simulink model "sm_car"  (R2025a)
settings: Solver=ode23t  StartTime=0.0  StopTime=400  MaxStep=0.4  RelTol=1e-3  AbsTol=1e-3  EnableMultiTasking=on
PreLoadFcn:
  | % Due to usability issue in Repeating Sequence block
  | warning('off','Simulink:Masking:Invalid');
  | 
  | % Eliminate unnecessary warnings in inactive variants
  | % Warnings generated only if you click through inactive variant
  | warning('off','MATLAB:nonExistentField');
  | warning('off','Simulink:Parameters:BlkParamUndefined');
PostLoadFcn:
  | set_param([bdroot '/Vehicle'],'popup_trailer','Off')
  | warning('off','sm:sli:setup:compile:LocalSolverNotSupported')
  | %sm_car_config_maneuver(bdroot,'WOT Braking');
  | sm_car_config_vehicle(bdroot,'false');
  | sm_car_config_logging(bdroot);
InitFcn:
  | sm_car_config_camera;
  | Vehicle = sm_car_vehcfg_checkConfig(Vehicle);
  | sm_car_check_tire_model(bdroot);
StartFcn:
  | tic;
StopFcn:
  | Elapsed_Sim_Time = toc;
  | % disp(['Elapsed Sim Time = ' num2str(Elapsed_Sim_Time)]);
undefined symbols (not defined in the file): Axle1D, AxleIn, Camera, Control, Driver, Free, Init, Maneuver, Pedal, RaceFix, RaceSpin, Scene, ShaftL1, ShaftL2, ShaftR1, ShaftR2, Soft, Stiff, Visual, X, xy_data_car_side, Y, Z
libraries: sm_lib x1546, nesl_utility x528, fl_lib x480, SimscapeFluids_lib x61, sdl_lib x49, simulink x29, ee_lib x7, simulink_extras x6, Linkage_Systems x4, Tire_1x2x x4, AntiRollBar_Systems x2, Linkage_Decoupled x2
(part 23 of 79)

== system sm_car/Vehicle/Vehicle/Chassis/Damper/Decoupled/Damper A1 Heave/Variable Endstop NL ==
  note: Sensing
  Ctrl : Inport
  Bumpstop : sdl_lib/Couplings & Drives/Springs & Dampers/Nonlinear Translational Spring  parameterization=sdl.enum.polynomialTLU.tlu  symmetry=sdl.enum.symmetry.twoSided  coefficient_vector=[100, 0, 10, 0, 1] N/m  tension_coefficient_vector=[100, 0, 10, 0, 1] N/m  compression_coefficient_vector=[1000, -10, 100, 0, 0] N/m  deformation_vector=xEndstop m  force_vector=fEndstop N  interp_method=simscape.enum.interpolation.linear  extrap_method=simscape.enum.extrapolation.linear  x_specify=on  x_priority=None  x=0 m  x_nominal_specify=off  x_nominal_value=1  x_nominal_unit=m
      settings: InternalSimscapePortConfiguration="{\"Bottom\":[],\"Left\":[{\"id\":\"R\",\"label\":\"R\",\"type\":\"foundation.mechanical.translational.translational\"}],\"Right\":[{\"id\":\"C\",\"label\":\"C\",\"type\":\"foundation.mechanical.translational.translational\"}],\"Top\":[]}"
  Damper : sdl_lib/Couplings & Drives/Springs & Dampers/Variable Translational Damper  Bmin=0 N*s/m
      settings: InternalSimscapePortConfiguration="{\"Bottom\":[],\"Left\":[{\"id\":\"B\",\"label\":\"B\",\"type\":\"input\"},{\"id\":\"R\",\"label\":\"R\",\"type\":\"foundation.mechanical.translational.translational\"}],\"Right\":[{\"id\":\"C\",\"label\":\"C\",\"type\":\"foundation.mechanical.translational.translational\"}],\"Top\":[]}"
  Force Bumpstop : fl_lib/Mechanical/Mechanical Sensors/Ideal Force Sensor
  Force Damper : fl_lib/Mechanical/Mechanical Sensors/Ideal Force Sensor
  Motion Damper : fl_lib/Mechanical/Mechanical Sensors/Ideal Translational Motion Sensor  reference=foundation.enum.MeasurementReference.difference  acceleration_port=false  velocity_port=true  position_port=true  offset=dam_x0 m
  PS-Simulink Converter : nesl_utility/PS-Simulink Converter  PhysicalDomain=network_engine_domain  SubClassName=ps_output  LeftPortType=input  RightPortType=output  PseudoPeriodic=off  Frequencies=[]  VectorFormat=1-D array  Unit=N  AffineConversion=off
  PS-Simulink Converter1 : nesl_utility/PS-Simulink Converter  PhysicalDomain=network_engine_domain  SubClassName=ps_output  LeftPortType=input  RightPortType=output  PseudoPeriodic=off  Frequencies=[]  VectorFormat=1-D array  Unit=N  AffineConversion=off
  PS-Simulink Converter2 : nesl_utility/PS-Simulink Converter  PhysicalDomain=network_engine_domain  SubClassName=ps_output  LeftPortType=input  RightPortType=output  PseudoPeriodic=off  Frequencies=[]  VectorFormat=1-D array  Unit=m/s  AffineConversion=off
  PS-Simulink Converter3 : nesl_utility/PS-Simulink Converter  PhysicalDomain=network_engine_domain  SubClassName=ps_output  LeftPortType=input  RightPortType=output  PseudoPeriodic=off  Frequencies=[]  VectorFormat=1-D array  Unit=m  AffineConversion=off
  Simulink-PS Converter : nesl_utility/Simulink-PS Converter  PhysicalDomain=network_engine_domain  SubClassName=ps_input  LeftPortType=input  RightPortType=output  PseudoPeriodic=off  Frequencies=[]  NoiseDistribution=none  NoiseParameters=[]  Unit=N*s/m  AffineConversion=off  FilteringAndDerivatives=provide  SimscapeFilterOrder=1  InputFilterTimeConstant=0.001  UdotUserProvided=0
  R : PMIOPort  Side=Left
  C : PMIOPort  Port=2  Side=Right
  Out Bus Element : Outport  VectorParamsAs1DForOutWhenUnconnected=off  PortName=meas  Element=FDamper
  Out Bus Element1 : Outport  VectorParamsAs1DForOutWhenUnconnected=off  PortName=meas  Element=FBumpstop
  Out Bus Element2 : Outport  VectorParamsAs1DForOutWhenUnconnected=off  PortName=meas  Element=xDamper
  Out Bus Element3 : Outport  VectorParamsAs1DForOutWhenUnconnected=off  PortName=meas  Element=vDamper
  wires:
  PS-Simulink Converter1/1 -> Out Bus Element1/1
  PS-Simulink Converter3/1 -> Out Bus Element2/1
  PS-Simulink Converter2/1 -> Out Bus Element3/1
  PS-Simulink Converter/1 -> Out Bus Element/1
  Ctrl/1 -> Simulink-PS Converter/1
  connections:
  Simulink-PS Converter/RConn1 -- Damper/LConn1
  R/RConn1 -- Motion Damper/LConn1 -- Bumpstop/LConn1 -- Damper/LConn2
  Force Damper/RConn1 -- Damper/RConn1
  Bumpstop/RConn1 -- Force Bumpstop/RConn1
  PS-Simulink Converter/LConn1 -- Force Damper/RConn2
  PS-Simulink Converter3/LConn1 -- Motion Damper/RConn3
  PS-Simulink Converter1/LConn1 -- Force Bumpstop/RConn2
  PS-Simulink Converter2/LConn1 -- Motion Damper/RConn2
  Force Damper/LConn1 -- C/RConn1 -- Force Bumpstop/LConn1 -- Motion Damper/RConn1

== system sm_car/Vehicle/Vehicle/Chassis/Damper/Decoupled/Damper A1 Roll/Force Endstop NL ==
  note: Sensing
  Ctrl : Inport
  Bumpstop : sdl_lib/Couplings & Drives/Springs & Dampers/Nonlinear Translational Spring  parameterization=sdl.enum.polynomialTLU.tlu  symmetry=sdl.enum.symmetry.twoSided  coefficient_vector=[100, 0, 10, 0, 1] N/m  tension_coefficient_vector=[100, 0, 10, 0, 1] N/m  compression_coefficient_vector=[1000, -10, 100, 0, 0] N/m  deformation_vector=xEndstop m  force_vector=fEndstop N  interp_method=simscape.enum.interpolation.linear  extrap_method=simscape.enum.extrapolation.linear  x_specify=on  x_priority=None  x=0 m  x_nominal_specify=off  x_nominal_value=1  x_nominal_unit=m
      settings: InternalSimscapePortConfiguration="{\"Bottom\":[],\"Left\":[{\"id\":\"R\",\"label\":\"R\",\"type\":\"foundation.mechanical.translational.translational\"}],\"Right\":[{\"id\":\"C\",\"label\":\"C\",\"type\":\"foundation.mechanical.translational.translational\"}],\"Top\":[]}"
  Force Source : fl_lib/Mechanical/Mechanical Sources/Ideal Force Source
  Force Bumpstop : fl_lib/Mechanical/Mechanical Sensors/Ideal Force Sensor
  Force Damper : fl_lib/Mechanical/Mechanical Sensors/Ideal Force Sensor
  Motion Damper : fl_lib/Mechanical/Mechanical Sensors/Ideal Translational Motion Sensor  reference=foundation.enum.MeasurementReference.difference  acceleration_port=false  velocity_port=true  position_port=true  offset=dam_x0 m
  PS-Simulink Converter : nesl_utility/PS-Simulink Converter  PhysicalDomain=network_engine_domain  SubClassName=ps_output  LeftPortType=input  RightPortType=output  PseudoPeriodic=off  Frequencies=[]  VectorFormat=1-D array  Unit=N  AffineConversion=off
  PS-Simulink Converter1 : nesl_utility/PS-Simulink Converter  PhysicalDomain=network_engine_domain  SubClassName=ps_output  LeftPortType=input  RightPortType=output  PseudoPeriodic=off  Frequencies=[]  VectorFormat=1-D array  Unit=N  AffineConversion=off
  PS-Simulink Converter2 : nesl_utility/PS-Simulink Converter  PhysicalDomain=network_engine_domain  SubClassName=ps_output  LeftPortType=input  RightPortType=output  PseudoPeriodic=off  Frequencies=[]  VectorFormat=1-D array  Unit=m/s  AffineConversion=off
  PS-Simulink Converter3 : nesl_utility/PS-Simulink Converter  PhysicalDomain=network_engine_domain  SubClassName=ps_output  LeftPortType=input  RightPortType=output  PseudoPeriodic=off  Frequencies=[]  VectorFormat=1-D array  Unit=m  AffineConversion=off
  Simulink-PS Converter : nesl_utility/Simulink-PS Converter  PhysicalDomain=network_engine_domain  SubClassName=ps_input  LeftPortType=input  RightPortType=output  PseudoPeriodic=off  Frequencies=[]  NoiseDistribution=none  NoiseParameters=[]  Unit=N  AffineConversion=off  FilteringAndDerivatives=filter  SimscapeFilterOrder=1  InputFilterTimeConstant=0.01  UdotUserProvided=0
  R : PMIOPort  Side=Left
  C : PMIOPort  Port=2  Side=Right
  Out Bus Element : Outport  VectorParamsAs1DForOutWhenUnconnected=off  PortName=meas  Element=FDamper
  Out Bus Element1 : Outport  VectorParamsAs1DForOutWhenUnconnected=off  PortName=meas  Element=FBumpstop
  Out Bus Element2 : Outport  VectorParamsAs1DForOutWhenUnconnected=off  PortName=meas  Element=xDamper
  Out Bus Element3 : Outport  VectorParamsAs1DForOutWhenUnconnected=off  PortName=meas  Element=vDamper
  wires:
  PS-Simulink Converter1/1 -> Out Bus Element1/1
  PS-Simulink Converter3/1 -> Out Bus Element2/1
  PS-Simulink Converter2/1 -> Out Bus Element3/1
  PS-Simulink Converter/1 -> Out Bus Element/1
  Ctrl/1 -> Simulink-PS Converter/1
  connections:
  Simulink-PS Converter/RConn1 -- Force Source/RConn1
  Force Source/RConn2 -- Bumpstop/LConn1 -- R/RConn1 -- Motion Damper/LConn1
  Force Source/LConn1 -- Force Damper/RConn1
  Bumpstop/RConn1 -- Force Bumpstop/RConn1
  PS-Simulink Converter/LConn1 -- Force Damper/RConn2
  PS-Simulink Converter3/LConn1 -- Motion Damper/RConn3
  PS-Simulink Converter1/LConn1 -- Force Bumpstop/RConn2
  PS-Simulink Converter2/LConn1 -- Motion Damper/RConn2
  Force Damper/LConn1 -- C/RConn1 -- Force Bumpstop/LConn1 -- Motion Damper/RConn1

== system sm_car/Vehicle/Vehicle/Chassis/Damper/Decoupled/Damper A1 Roll/Linear ==
  note: Sensing
  Ctrl : Inport
  Bumpstop : fl_lib/Mechanical/Translational Elements/Translational Hard Stop  upper_bnd=bs_lim_upper m  lower_bnd=bs_lim_lower m  model=1  stiff_up=bs_k_upper N/m  stiff_low=bs_k_lower N/m  D_up=bs_b_upper N/(m/s)  D_low=bs_b_lower N/(m/s)  transition=bs_region m  coeff_rest=0.7  v_tol=0.001 m/s  f_tol=0.001 N  v_specify=off  v_priority=None  v=0 m/s  v_nominal_specify=off  v_nominal_value=1  v_nominal_unit=m/s  f_specify=off  f_priority=None  f=0 N  f_nominal_specify=off  f_nominal_value=1  f_nominal_unit=N  x_specify=off  x_priority=High  x=0 m  x_nominal_specify=off  x_nominal_value=1  x_nominal_unit=m  M_specify=off  M_priority=None  M=0
  Damper : fl_lib/Mechanical/Translational Elements/Translational Damper  D=dam_b N/(m/s)  v_specify=off  v_priority=None  v=0 m/s  v_nominal_specify=off  v_nominal_value=1  v_nominal_unit=m/s  f_specify=off  f_priority=None  f=0 N  f_nominal_specify=off  f_nominal_value=1  f_nominal_unit=N
  Force Bumpstop : fl_lib/Mechanical/Mechanical Sensors/Ideal Force Sensor
  Force Damper : fl_lib/Mechanical/Mechanical Sensors/Ideal Force Sensor
  Motion Damper : fl_lib/Mechanical/Mechanical Sensors/Ideal Translational Motion Sensor  reference=foundation.enum.MeasurementReference.difference  acceleration_port=false  velocity_port=true  position_port=true  offset=dam_x0 m
  PS-Simulink Converter : nesl_utility/PS-Simulink Converter  PhysicalDomain=network_engine_domain  SubClassName=ps_output  LeftPortType=input  RightPortType=output  PseudoPeriodic=off  Frequencies=[]  VectorFormat=1-D array  Unit=N  AffineConversion=off
  PS-Simulink Converter1 : nesl_utility/PS-Simulink Converter  PhysicalDomain=network_engine_domain  SubClassName=ps_output  LeftPortType=input  RightPortType=output  PseudoPeriodic=off  Frequencies=[]  VectorFormat=1-D array  Unit=N  AffineConversion=off
  PS-Simulink Converter2 : nesl_utility/PS-Simulink Converter  PhysicalDomain=network_engine_domain  SubClassName=ps_output  LeftPortType=input  RightPortType=output  PseudoPeriodic=off  Frequencies=[]  VectorFormat=1-D array  Unit=m/s  AffineConversion=off
  PS-Simulink Converter3 : nesl_utility/PS-Simulink Converter  PhysicalDomain=network_engine_domain  SubClassName=ps_output  LeftPortType=input  RightPortType=output  PseudoPeriodic=off  Frequencies=[]  VectorFormat=1-D array  Unit=m  AffineConversion=off
  Terminator : Terminator
  R : PMIOPort  Side=Left
  C : PMIOPort  Port=2  Side=Right
  Out Bus Element : Outport  VectorParamsAs1DForOutWhenUnconnected=off  PortName=meas  Element=FDamper
  Out Bus Element1 : Outport  VectorParamsAs1DForOutWhenUnconnected=off  PortName=meas  Element=FBumpstop
  Out Bus Element2 : Outport  VectorParamsAs1DForOutWhenUnconnected=off  PortName=meas  Element=xDamper
  Out Bus Element3 : Outport  VectorParamsAs1DForOutWhenUnconnected=off  PortName=meas  Element=vDamper
  wires:
  PS-Simulink Converter1/1 -> Out Bus Element1/1
  PS-Simulink Converter3/1 -> Out Bus Element2/1
  PS-Simulink Converter2/1 -> Out Bus Element3/1
  PS-Simulink Converter/1 -> Out Bus Element/1
  Ctrl/1 -> Terminator/1
  connections:
  R/RConn1 -- Motion Damper/LConn1 -- Bumpstop/LConn1 -- Damper/LConn1
  Force Damper/RConn1 -- Damper/RConn1
  Force Bumpstop/RConn1 -- Bumpstop/RConn1
  PS-Simulink Converter/LConn1 -- Force Damper/RConn2
  PS-Simulink Converter3/LConn1 -- Motion Damper/RConn3
  PS-Simulink Converter1/LConn1 -- Force Bumpstop/RConn2
  PS-Simulink Converter2/LConn1 -- Motion Damper/RConn2
  Force Damper/LConn1 -- C/RConn1 -- Force Bumpstop/LConn1 -- Motion Damper/RConn1

== system sm_car/Vehicle/Vehicle/Chassis/Damper/Decoupled/Damper A1 Roll/None ==
  note: Sensor inserted simply to ensure
      | all blocks are connected to a network
  Ctrl : Inport
  Constant{1..4} (4 alike) : Constant  Value=0
  Ideal Translational Motion Sensor : fl_lib/Mechanical/Mechanical Sensors/Ideal Translational Motion Sensor  reference=foundation.enum.MeasurementReference.difference  acceleration_port=false  velocity_port=true  position_port=true  offset=0 m
  PS-Simulink Converter2 : nesl_utility/PS-Simulink Converter  PhysicalDomain=network_engine_domain  SubClassName=ps_output  LeftPortType=input  RightPortType=output  PseudoPeriodic=off  Frequencies=[]  VectorFormat=1-D array  Unit=1  AffineConversion=off
  PS-Simulink Converter3 : nesl_utility/PS-Simulink Converter  PhysicalDomain=network_engine_domain  SubClassName=ps_output  LeftPortType=input  RightPortType=output  PseudoPeriodic=off  Frequencies=[]  VectorFormat=1-D array  Unit=1  AffineConversion=off
  Terminator : Terminator
  Terminator1 : Terminator
  Terminator2 : Terminator
  R : PMIOPort  Side=Left
  C : PMIOPort  Port=2  Side=Right
  Out Bus Element : Outport  VectorParamsAs1DForOutWhenUnconnected=off  PortName=meas  Element=FDamper
  Out Bus Element1 : Outport  VectorParamsAs1DForOutWhenUnconnected=off  PortName=meas  Element=FBumpstop
  Out Bus Element2 : Outport  VectorParamsAs1DForOutWhenUnconnected=off  PortName=meas  Element=xDamper
  Out Bus Element3 : Outport  VectorParamsAs1DForOutWhenUnconnected=off  PortName=meas  Element=vDamper
  wires:
  PS-Simulink Converter2/1 -> Terminator1/1
  PS-Simulink Converter3/1 -> Terminator2/1
  Constant2/1 -> Out Bus Element1/1
  Constant4/1 -> Out Bus Element2/1
  Constant3/1 -> Out Bus Element3/1
  Constant1/1 -> Out Bus Element/1
  Ctrl/1 -> Terminator/1
  connections:
  C/RConn1 -- Ideal Translational Motion Sensor/RConn1
  R/RConn1 -- Ideal Translational Motion Sensor/LConn1
  PS-Simulink Converter3/LConn1 -- Ideal Translational Motion Sensor/RConn3
  Ideal Translational Motion Sensor/RConn2 -- PS-Simulink Converter2/LConn1

== system sm_car/Vehicle/Vehicle/Chassis/Damper/Decoupled/Damper A1 Roll/Nonlinear ==
  note: Sensing
  Ctrl : Inport
  Bumpstop : fl_lib/Mechanical/Translational Elements/Translational Hard Stop  upper_bnd=bs_lim_upper m  lower_bnd=bs_lim_lower m  model=1  stiff_up=bs_k_upper N/m  stiff_low=bs_k_lower N/m  D_up=bs_b_upper N/(m/s)  D_low=bs_b_lower N/(m/s)  transition=bs_region m  coeff_rest=0.7  v_tol=0.001 m/s  f_tol=0.001 N  v_specify=off  v_priority=None  v=0 m/s  v_nominal_specify=off  v_nominal_value=1  v_nominal_unit=m/s  f_specify=off  f_priority=None  f=0 N  f_nominal_specify=off  f_nominal_value=1  f_nominal_unit=N  x_specify=off  x_priority=High  x=0 m  x_nominal_specify=off  x_nominal_value=1  x_nominal_unit=m  M_specify=off  M_priority=None  M=0
  Damper : sdl_lib/Couplings & Drives/Springs & Dampers/Nonlinear Translational Damper  parameterization=2  symmetry=1  coefficient_vector=[10, 0, 1, 0, .1] N/(m/s)  extension_coefficient_vector=[10, 0, 1, 0, .1] N/(m/s)  contraction_coefficient_vector=[100, -1, 10, 0, 0] N/(m/s)  velocity_vector=velocity_vector m/s  force_vector=force_vector N  interp_method=simscape.enum.interpolation.linear  extrap_method=simscape.enum.extrapolation.linear
      settings: InternalSimscapePortConfiguration="{\"Bottom\":[],\"Left\":[{\"id\":\"R\",\"label\":\"R\",\"type\":\"foundation.mechanical.translational.translational\"}],\"Right\":[{\"id\":\"C\",\"label\":\"C\",\"type\":\"foundation.mechanical.translational.translational\"}],\"Top\":[]}"
  Force Bumpstop : fl_lib/Mechanical/Mechanical Sensors/Ideal Force Sensor
  Force Damper : fl_lib/Mechanical/Mechanical Sensors/Ideal Force Sensor
  Motion Damper : fl_lib/Mechanical/Mechanical Sensors/Ideal Translational Motion Sensor  reference=foundation.enum.MeasurementReference.difference  acceleration_port=false  velocity_port=true  position_port=true  offset=dam_x0 m
  PS-Simulink Converter : nesl_utility/PS-Simulink Converter  PhysicalDomain=network_engine_domain  SubClassName=ps_output  LeftPortType=input  RightPortType=output  PseudoPeriodic=off  Frequencies=[]  VectorFormat=1-D array  Unit=N  AffineConversion=off
  PS-Simulink Converter1 : nesl_utility/PS-Simulink Converter  PhysicalDomain=network_engine_domain  SubClassName=ps_output  LeftPortType=input  RightPortType=output  PseudoPeriodic=off  Frequencies=[]  VectorFormat=1-D array  Unit=N  AffineConversion=off
  PS-Simulink Converter2 : nesl_utility/PS-Simulink Converter  PhysicalDomain=network_engine_domain  SubClassName=ps_output  LeftPortType=input  RightPortType=output  PseudoPeriodic=off  Frequencies=[]  VectorFormat=1-D array  Unit=m/s  AffineConversion=off
  PS-Simulink Converter3 : nesl_utility/PS-Simulink Converter  PhysicalDomain=network_engine_domain  SubClassName=ps_output  LeftPortType=input  RightPortType=output  PseudoPeriodic=off  Frequencies=[]  VectorFormat=1-D array  Unit=m  AffineConversion=off
  Terminator : Terminator
  R : PMIOPort  Side=Left
  C : PMIOPort  Port=2  Side=Right
  Out Bus Element : Outport  VectorParamsAs1DForOutWhenUnconnected=off  PortName=meas  Element=FDamper
  Out Bus Element1 : Outport  VectorParamsAs1DForOutWhenUnconnected=off  PortName=meas  Element=FBumpstop
  Out Bus Element2 : Outport  VectorParamsAs1DForOutWhenUnconnected=off  PortName=meas  Element=xDamper
  Out Bus Element3 : Outport  VectorParamsAs1DForOutWhenUnconnected=off  PortName=meas  Element=vDamper
  wires:
  Ctrl/1 -> Terminator/1
  PS-Simulink Converter/1 -> Out Bus Element/1
  PS-Simulink Converter2/1 -> Out Bus Element3/1
  PS-Simulink Converter3/1 -> Out Bus Element2/1
  PS-Simulink Converter1/1 -> Out Bus Element1/1
  connections:
  Motion Damper/RConn1 -- Force Bumpstop/LConn1 -- C/RConn1 -- Force Damper/LConn1
  PS-Simulink Converter2/LConn1 -- Motion Damper/RConn2
  PS-Simulink Converter1/LConn1 -- Force Bumpstop/RConn2
  PS-Simulink Converter3/LConn1 -- Motion Damper/RConn3
  PS-Simulink Converter/LConn1 -- Force Damper/RConn2
  Force Bumpstop/RConn1 -- Bumpstop/RConn1
  Damper/RConn1 -- Force Damper/RConn1
  Bumpstop/LConn1 -- Motion Damper/LConn1 -- R/RConn1 -- Damper/LConn1

== system sm_car/Vehicle/Vehicle/Chassis/Damper/Decoupled/Damper A1 Roll/Nonlinear Endstop NL ==
  note: Sensing
  Ctrl : Inport
  Bumpstop : sdl_lib/Couplings & Drives/Springs & Dampers/Nonlinear Translational Spring  parameterization=sdl.enum.polynomialTLU.tlu  symmetry=sdl.enum.symmetry.twoSided  coefficient_vector=[100, 0, 10, 0, 1] N/m  tension_coefficient_vector=[100, 0, 10, 0, 1] N/m  compression_coefficient_vector=[1000, -10, 100, 0, 0] N/m  deformation_vector=xEndstop m  force_vector=fEndstop N  interp_method=simscape.enum.interpolation.linear  extrap_method=simscape.enum.extrapolation.linear  x_specify=on  x_priority=None  x=0 m  x_nominal_specify=off  x_nominal_value=1  x_nominal_unit=m
      settings: InternalSimscapePortConfiguration="{\"Bottom\":[],\"Left\":[{\"id\":\"R\",\"label\":\"R\",\"type\":\"foundation.mechanical.translational.translational\"}],\"Right\":[{\"id\":\"C\",\"label\":\"C\",\"type\":\"foundation.mechanical.translational.translational\"}],\"Top\":[]}"
  Damper : sdl_lib/Couplings & Drives/Springs & Dampers/Nonlinear Translational Damper  parameterization=2  symmetry=1  coefficient_vector=[10, 0, 1, 0, .1] N/(m/s)  extension_coefficient_vector=[10, 0, 1, 0, .1] N/(m/s)  contraction_coefficient_vector=[100, -1, 10, 0, 0] N/(m/s)  velocity_vector=velocity_vector m/s  force_vector=force_vector N  interp_method=simscape.enum.interpolation.linear  extrap_method=simscape.enum.extrapolation.linear
      settings: InternalSimscapePortConfiguration="{\"Bottom\":[],\"Left\":[{\"id\":\"R\",\"label\":\"R\",\"type\":\"foundation.mechanical.translational.translational\"}],\"Right\":[{\"id\":\"C\",\"label\":\"C\",\"type\":\"foundation.mechanical.translational.translational\"}],\"Top\":[]}"
  Force Bumpstop : fl_lib/Mechanical/Mechanical Sensors/Ideal Force Sensor
  Force Damper : fl_lib/Mechanical/Mechanical Sensors/Ideal Force Sensor
  Motion Damper : fl_lib/Mechanical/Mechanical Sensors/Ideal Translational Motion Sensor  reference=foundation.enum.MeasurementReference.difference  acceleration_port=false  velocity_port=true  position_port=true  offset=dam_x0 m
  PS-Simulink Converter : nesl_utility/PS-Simulink Converter  PhysicalDomain=network_engine_domain  SubClassName=ps_output  LeftPortType=input  RightPortType=output  PseudoPeriodic=off  Frequencies=[]  VectorFormat=1-D array  Unit=N  AffineConversion=off
  PS-Simulink Converter1 : nesl_utility/PS-Simulink Converter  PhysicalDomain=network_engine_domain  SubClassName=ps_output  LeftPortType=input  RightPortType=output  PseudoPeriodic=off  Frequencies=[]  VectorFormat=1-D array  Unit=N  AffineConversion=off
  PS-Simulink Converter2 : nesl_utility/PS-Simulink Converter  PhysicalDomain=network_engine_domain  SubClassName=ps_output  LeftPortType=input  RightPortType=output  PseudoPeriodic=off  Frequencies=[]  VectorFormat=1-D array  Unit=m/s  AffineConversion=off
  PS-Simulink Converter3 : nesl_utility/PS-Simulink Converter  PhysicalDomain=network_engine_domain  SubClassName=ps_output  LeftPortType=input  RightPortType=output  PseudoPeriodic=off  Frequencies=[]  VectorFormat=1-D array  Unit=m  AffineConversion=off
  Terminator : Terminator
  R : PMIOPort  Side=Left
  C : PMIOPort  Port=2  Side=Right
  Out Bus Element : Outport  VectorParamsAs1DForOutWhenUnconnected=off  PortName=meas  Element=FDamper
  Out Bus Element1 : Outport  VectorParamsAs1DForOutWhenUnconnected=off  PortName=meas  Element=FBumpstop
  Out Bus Element2 : Outport  VectorParamsAs1DForOutWhenUnconnected=off  PortName=meas  Element=xDamper
  Out Bus Element3 : Outport  VectorParamsAs1DForOutWhenUnconnected=off  PortName=meas  Element=vDamper
  wires:
  Ctrl/1 -> Terminator/1
  PS-Simulink Converter/1 -> Out Bus Element/1
  PS-Simulink Converter2/1 -> Out Bus Element3/1
  PS-Simulink Converter3/1 -> Out Bus Element2/1
  PS-Simulink Converter1/1 -> Out Bus Element1/1
  connections:
  Motion Damper/RConn1 -- Force Bumpstop/LConn1 -- C/RConn1 -- Force Damper/LConn1
  PS-Simulink Converter2/LConn1 -- Motion Damper/RConn2
  PS-Simulink Converter1/LConn1 -- Force Bumpstop/RConn2
  PS-Simulink Converter3/LConn1 -- Motion Damper/RConn3
  PS-Simulink Converter/LConn1 -- Force Damper/RConn2
  Force Bumpstop/RConn1 -- Bumpstop/RConn1
  Damper/RConn1 -- Force Damper/RConn1
  Motion Damper/LConn1 -- R/RConn1 -- Bumpstop/LConn1 -- Damper/LConn1

== system sm_car/Vehicle/Vehicle/Chassis/Damper/Decoupled/Damper A1 Roll/Variable ==
  note: Sensing
  Ctrl : Inport
  Bumpstop : fl_lib/Mechanical/Translational Elements/Translational Hard Stop  upper_bnd=bs_lim_upper m  lower_bnd=bs_lim_lower m  model=1  stiff_up=bs_k_upper N/m  stiff_low=bs_k_lower N/m  D_up=bs_b_upper N/(m/s)  D_low=bs_b_lower N/(m/s)  transition=bs_region m  coeff_rest=0.7  v_tol=0.001 m/s  f_tol=0.001 N  v_specify=off  v_priority=None  v=0 m/s  v_nominal_specify=off  v_nominal_value=1  v_nominal_unit=m/s  f_specify=off  f_priority=None  f=0 N  f_nominal_specify=off  f_nominal_value=1  f_nominal_unit=N  x_specify=off  x_priority=High  x=0 m  x_nominal_specify=off  x_nominal_value=1  x_nominal_unit=m  M_specify=off  M_priority=None  M=0
  Damper : sdl_lib/Couplings & Drives/Springs & Dampers/Variable Translational Damper  Bmin=0 N*s/m
      settings: InternalSimscapePortConfiguration="{\"Bottom\":[],\"Left\":[{\"id\":\"B\",\"label\":\"B\",\"type\":\"input\"},{\"id\":\"R\",\"label\":\"R\",\"type\":\"foundation.mechanical.translational.translational\"}],\"Right\":[{\"id\":\"C\",\"label\":\"C\",\"type\":\"foundation.mechanical.translational.translational\"}],\"Top\":[]}"
  Force Bumpstop : fl_lib/Mechanical/Mechanical Sensors/Ideal Force Sensor
  Force Damper : fl_lib/Mechanical/Mechanical Sensors/Ideal Force Sensor
  Motion Damper : fl_lib/Mechanical/Mechanical Sensors/Ideal Translational Motion Sensor  reference=foundation.enum.MeasurementReference.difference  acceleration_port=false  velocity_port=true  position_port=true  offset=dam_x0 m
  PS-Simulink Converter : nesl_utility/PS-Simulink Converter  PhysicalDomain=network_engine_domain  SubClassName=ps_output  LeftPortType=input  RightPortType=output  PseudoPeriodic=off  Frequencies=[]  VectorFormat=1-D array  Unit=N  AffineConversion=off
  PS-Simulink Converter1 : nesl_utility/PS-Simulink Converter  PhysicalDomain=network_engine_domain  SubClassName=ps_output  LeftPortType=input  RightPortType=output  PseudoPeriodic=off  Frequencies=[]  VectorFormat=1-D array  Unit=N  AffineConversion=off
  PS-Simulink Converter2 : nesl_utility/PS-Simulink Converter  PhysicalDomain=network_engine_domain  SubClassName=ps_output  LeftPortType=input  RightPortType=output  PseudoPeriodic=off  Frequencies=[]  VectorFormat=1-D array  Unit=m/s  AffineConversion=off
  PS-Simulink Converter3 : nesl_utility/PS-Simulink Converter  PhysicalDomain=network_engine_domain  SubClassName=ps_output  LeftPortType=input  RightPortType=output  PseudoPeriodic=off  Frequencies=[]  VectorFormat=1-D array  Unit=m  AffineConversion=off
  Simulink-PS Converter : nesl_utility/Simulink-PS Converter  PhysicalDomain=network_engine_domain  SubClassName=ps_input  LeftPortType=input  RightPortType=output  PseudoPeriodic=off  Frequencies=[]  NoiseDistribution=none  NoiseParameters=[]  Unit=N*s/m  AffineConversion=off  FilteringAndDerivatives=provide  SimscapeFilterOrder=1  InputFilterTimeConstant=0.001  UdotUserProvided=0
  R : PMIOPort  Side=Left
  C : PMIOPort  Port=2  Side=Right
  Out Bus Element : Outport  VectorParamsAs1DForOutWhenUnconnected=off  PortName=meas  Element=FDamper
  Out Bus Element1 : Outport  VectorParamsAs1DForOutWhenUnconnected=off  PortName=meas  Element=FBumpstop
  Out Bus Element2 : Outport  VectorParamsAs1DForOutWhenUnconnected=off  PortName=meas  Element=xDamper
  Out Bus Element3 : Outport  VectorParamsAs1DForOutWhenUnconnected=off  PortName=meas  Element=vDamper
  wires:
  PS-Simulink Converter1/1 -> Out Bus Element1/1
  PS-Simulink Converter3/1 -> Out Bus Element2/1
  PS-Simulink Converter2/1 -> Out Bus Element3/1
  PS-Simulink Converter/1 -> Out Bus Element/1
  Ctrl/1 -> Simulink-PS Converter/1
  connections:
  Simulink-PS Converter/RConn1 -- Damper/LConn1
  R/RConn1 -- Motion Damper/LConn1 -- Damper/LConn2 -- Bumpstop/LConn1
  Force Damper/RConn1 -- Damper/RConn1
  Force Bumpstop/RConn1 -- Bumpstop/RConn1
  PS-Simulink Converter/LConn1 -- Force Damper/RConn2
  PS-Simulink Converter3/LConn1 -- Motion Damper/RConn3
  PS-Simulink Converter1/LConn1 -- Force Bumpstop/RConn2
  PS-Simulink Converter2/LConn1 -- Motion Damper/RConn2
  Force Damper/LConn1 -- C/RConn1 -- Force Bumpstop/LConn1 -- Motion Damper/RConn1

== system sm_car/Vehicle/Vehicle/Chassis/Damper/Decoupled/Damper A1 Roll/Variable Endstop NL ==
  note: Sensing
  Ctrl : Inport
  Bumpstop : sdl_lib/Couplings & Drives/Springs & Dampers/Nonlinear Translational Spring  parameterization=sdl.enum.polynomialTLU.tlu  symmetry=sdl.enum.symmetry.twoSided  coefficient_vector=[100, 0, 10, 0, 1] N/m  tension_coefficient_vector=[100, 0, 10, 0, 1] N/m  compression_coefficient_vector=[1000, -10, 100, 0, 0] N/m  deformation_vector=xEndstop m  force_vector=fEndstop N  interp_method=simscape.enum.interpolation.linear  extrap_method=simscape.enum.extrapolation.linear  x_specify=on  x_priority=None  x=0 m  x_nominal_specify=off  x_nominal_value=1  x_nominal_unit=m
      settings: InternalSimscapePortConfiguration="{\"Bottom\":[],\"Left\":[{\"id\":\"R\",\"label\":\"R\",\"type\":\"foundation.mechanical.translational.translational\"}],\"Right\":[{\"id\":\"C\",\"label\":\"C\",\"type\":\"foundation.mechanical.translational.translational\"}],\"Top\":[]}"
  Damper : sdl_lib/Couplings & Drives/Springs & Dampers/Variable Translational Damper  Bmin=0 N*s/m
      settings: InternalSimscapePortConfiguration="{\"Bottom\":[],\"Left\":[{\"id\":\"B\",\"label\":\"B\",\"type\":\"input\"},{\"id\":\"R\",\"label\":\"R\",\"type\":\"foundation.mechanical.translational.translational\"}],\"Right\":[{\"id\":\"C\",\"label\":\"C\",\"type\":\"foundation.mechanical.translational.translational\"}],\"Top\":[]}"
  Force Bumpstop : fl_lib/Mechanical/Mechanical Sensors/Ideal Force Sensor
  Force Damper : fl_lib/Mechanical/Mechanical Sensors/Ideal Force Sensor
  Motion Damper : fl_lib/Mechanical/Mechanical Sensors/Ideal Translational Motion Sensor  reference=foundation.enum.MeasurementReference.difference  acceleration_port=false  velocity_port=true  position_port=true  offset=dam_x0 m
  PS-Simulink Converter : nesl_utility/PS-Simulink Converter  PhysicalDomain=network_engine_domain  SubClassName=ps_output  LeftPortType=input  RightPortType=output  PseudoPeriodic=off  Frequencies=[]  VectorFormat=1-D array  Unit=N  AffineConversion=off
  PS-Simulink Converter1 : nesl_utility/PS-Simulink Converter  PhysicalDomain=network_engine_domain  SubClassName=ps_output  LeftPortType=input  RightPortType=output  PseudoPeriodic=off  Frequencies=[]  VectorFormat=1-D array  Unit=N  AffineConversion=off
  PS-Simulink Converter2 : nesl_utility/PS-Simulink Converter  PhysicalDomain=network_engine_domain  SubClassName=ps_output  LeftPortType=input  RightPortType=output  PseudoPeriodic=off  Frequencies=[]  VectorFormat=1-D array  Unit=m/s  AffineConversion=off
  PS-Simulink Converter3 : nesl_utility/PS-Simulink Converter  PhysicalDomain=network_engine_domain  SubClassName=ps_output  LeftPortType=input  RightPortType=output  PseudoPeriodic=off  Frequencies=[]  VectorFormat=1-D array  Unit=m  AffineConversion=off
  Simulink-PS Converter : nesl_utility/Simulink-PS Converter  PhysicalDomain=network_engine_domain  SubClassName=ps_input  LeftPortType=input  RightPortType=output  PseudoPeriodic=off  Frequencies=[]  NoiseDistribution=none  NoiseParameters=[]  Unit=N*s/m  AffineConversion=off  FilteringAndDerivatives=provide  SimscapeFilterOrder=1  InputFilterTimeConstant=0.001  UdotUserProvided=0
  R : PMIOPort  Side=Left
  C : PMIOPort  Port=2  Side=Right
  Out Bus Element : Outport  VectorParamsAs1DForOutWhenUnconnected=off  PortName=meas  Element=FDamper
  Out Bus Element1 : Outport  VectorParamsAs1DForOutWhenUnconnected=off  PortName=meas  Element=FBumpstop
  Out Bus Element2 : Outport  VectorParamsAs1DForOutWhenUnconnected=off  PortName=meas  Element=xDamper
  Out Bus Element3 : Outport  VectorParamsAs1DForOutWhenUnconnected=off  PortName=meas  Element=vDamper
  wires:
  PS-Simulink Converter1/1 -> Out Bus Element1/1
  PS-Simulink Converter3/1 -> Out Bus Element2/1
  PS-Simulink Converter2/1 -> Out Bus Element3/1
  PS-Simulink Converter/1 -> Out Bus Element/1
  Ctrl/1 -> Simulink-PS Converter/1
  connections:
  Simulink-PS Converter/RConn1 -- Damper/LConn1
  R/RConn1 -- Motion Damper/LConn1 -- Bumpstop/LConn1 -- Damper/LConn2
  Force Damper/RConn1 -- Damper/RConn1
  Bumpstop/RConn1 -- Force Bumpstop/RConn1
  PS-Simulink Converter/LConn1 -- Force Damper/RConn2
  PS-Simulink Converter3/LConn1 -- Motion Damper/RConn3
  PS-Simulink Converter1/LConn1 -- Force Bumpstop/RConn2
  PS-Simulink Converter2/LConn1 -- Motion Damper/RConn2
  Force Damper/LConn1 -- C/RConn1 -- Force Bumpstop/LConn1 -- Motion Damper/RConn1

== system sm_car/Vehicle/Vehicle/Chassis/Damper/Decoupled/Damper A2 Heave/Force Endstop NL ==
  note: Sensing
  Ctrl : Inport
  Bumpstop : sdl_lib/Couplings & Drives/Springs & Dampers/Nonlinear Translational Spring  parameterization=sdl.enum.polynomialTLU.tlu  symmetry=sdl.enum.symmetry.twoSided  coefficient_vector=[100, 0, 10, 0, 1] N/m  tension_coefficient_vector=[100, 0, 10, 0, 1] N/m  compression_coefficient_vector=[1000, -10, 100, 0, 0] N/m  deformation_vector=xEndstop m  force_vector=fEndstop N  interp_method=simscape.enum.interpolation.linear  extrap_method=simscape.enum.extrapolation.linear  x_specify=on  x_priority=None  x=0 m  x_nominal_specify=off  x_nominal_value=1  x_nominal_unit=m
      settings: InternalSimscapePortConfiguration="{\"Bottom\":[],\"Left\":[{\"id\":\"R\",\"label\":\"R\",\"type\":\"foundation.mechanical.translational.translational\"}],\"Right\":[{\"id\":\"C\",\"label\":\"C\",\"type\":\"foundation.mechanical.translational.translational\"}],\"Top\":[]}"
  Force Source : fl_lib/Mechanical/Mechanical Sources/Ideal Force Source
  Force Bumpstop : fl_lib/Mechanical/Mechanical Sensors/Ideal Force Sensor
  Force Damper : fl_lib/Mechanical/Mechanical Sensors/Ideal Force Sensor
  Motion Damper : fl_lib/Mechanical/Mechanical Sensors/Ideal Translational Motion Sensor  reference=foundation.enum.MeasurementReference.difference  acceleration_port=false  velocity_port=true  position_port=true  offset=dam_x0 m
  PS-Simulink Converter : nesl_utility/PS-Simulink Converter  PhysicalDomain=network_engine_domain  SubClassName=ps_output  LeftPortType=input  RightPortType=output  PseudoPeriodic=off  Frequencies=[]  VectorFormat=1-D array  Unit=N  AffineConversion=off
  PS-Simulink Converter1 : nesl_utility/PS-Simulink Converter  PhysicalDomain=network_engine_domain  SubClassName=ps_output  LeftPortType=input  RightPortType=output  PseudoPeriodic=off  Frequencies=[]  VectorFormat=1-D array  Unit=N  AffineConversion=off
  PS-Simulink Converter2 : nesl_utility/PS-Simulink Converter  PhysicalDomain=network_engine_domain  SubClassName=ps_output  LeftPortType=input  RightPortType=output  PseudoPeriodic=off  Frequencies=[]  VectorFormat=1-D array  Unit=m/s  AffineConversion=off
  PS-Simulink Converter3 : nesl_utility/PS-Simulink Converter  PhysicalDomain=network_engine_domain  SubClassName=ps_output  LeftPortType=input  RightPortType=output  PseudoPeriodic=off  Frequencies=[]  VectorFormat=1-D array  Unit=m  AffineConversion=off
  Simulink-PS Converter : nesl_utility/Simulink-PS Converter  PhysicalDomain=network_engine_domain  SubClassName=ps_input  LeftPortType=input  RightPortType=output  PseudoPeriodic=off  Frequencies=[]  NoiseDistribution=none  NoiseParameters=[]  Unit=N  AffineConversion=off  FilteringAndDerivatives=filter  SimscapeFilterOrder=1  InputFilterTimeConstant=0.01  UdotUserProvided=0
  R : PMIOPort  Side=Left
  C : PMIOPort  Port=2  Side=Right
  Out Bus Element : Outport  VectorParamsAs1DForOutWhenUnconnected=off  PortName=meas  Element=FDamper
  Out Bus Element1 : Outport  VectorParamsAs1DForOutWhenUnconnected=off  PortName=meas  Element=FBumpstop
  Out Bus Element2 : Outport  VectorParamsAs1DForOutWhenUnconnected=off  PortName=meas  Element=xDamper
  Out Bus Element3 : Outport  VectorParamsAs1DForOutWhenUnconnected=off  PortName=meas  Element=vDamper
  wires:
  PS-Simulink Converter1/1 -> Out Bus Element1/1
  PS-Simulink Converter3/1 -> Out Bus Element2/1
  PS-Simulink Converter2/1 -> Out Bus Element3/1
  PS-Simulink Converter/1 -> Out Bus Element/1
  Ctrl/1 -> Simulink-PS Converter/1
  connections:
  Simulink-PS Converter/RConn1 -- Force Source/RConn1
  Force Source/RConn2 -- Bumpstop/LConn1 -- R/RConn1 -- Motion Damper/LConn1
  Force Source/LConn1 -- Force Damper/RConn1
  Bumpstop/RConn1 -- Force Bumpstop/RConn1
  PS-Simulink Converter/LConn1 -- Force Damper/RConn2
  PS-Simulink Converter3/LConn1 -- Motion Damper/RConn3
  PS-Simulink Converter1/LConn1 -- Force Bumpstop/RConn2
  PS-Simulink Converter2/LConn1 -- Motion Damper/RConn2
  Force Damper/LConn1 -- C/RConn1 -- Force Bumpstop/LConn1 -- Motion Damper/RConn1

== system sm_car/Vehicle/Vehicle/Chassis/Damper/Decoupled/Damper A2 Heave/Linear ==
  note: Sensing
  Ctrl : Inport
  Bumpstop : fl_lib/Mechanical/Translational Elements/Translational Hard Stop  upper_bnd=bs_lim_upper m  lower_bnd=bs_lim_lower m  model=1  stiff_up=bs_k_upper N/m  stiff_low=bs_k_lower N/m  D_up=bs_b_upper N/(m/s)  D_low=bs_b_lower N/(m/s)  transition=bs_region m  coeff_rest=0.7  v_tol=0.001 m/s  f_tol=0.001 N  v_specify=off  v_priority=None  v=0 m/s  v_nominal_specify=off  v_nominal_value=1  v_nominal_unit=m/s  f_specify=off  f_priority=None  f=0 N  f_nominal_specify=off  f_nominal_value=1  f_nominal_unit=N  x_specify=off  x_priority=High  x=0 m  x_nominal_specify=off  x_nominal_value=1  x_nominal_unit=m  M_specify=off  M_priority=None  M=0
  Damper : fl_lib/Mechanical/Translational Elements/Translational Damper  D=dam_b N/(m/s)  v_specify=off  v_priority=None  v=0 m/s  v_nominal_specify=off  v_nominal_value=1  v_nominal_unit=m/s  f_specify=off  f_priority=None  f=0 N  f_nominal_specify=off  f_nominal_value=1  f_nominal_unit=N
  Force Bumpstop : fl_lib/Mechanical/Mechanical Sensors/Ideal Force Sensor
  Force Damper : fl_lib/Mechanical/Mechanical Sensors/Ideal Force Sensor
  Motion Damper : fl_lib/Mechanical/Mechanical Sensors/Ideal Translational Motion Sensor  reference=foundation.enum.MeasurementReference.difference  acceleration_port=false  velocity_port=true  position_port=true  offset=dam_x0 m
  PS-Simulink Converter : nesl_utility/PS-Simulink Converter  PhysicalDomain=network_engine_domain  SubClassName=ps_output  LeftPortType=input  RightPortType=output  PseudoPeriodic=off  Frequencies=[]  VectorFormat=1-D array  Unit=N  AffineConversion=off
  PS-Simulink Converter1 : nesl_utility/PS-Simulink Converter  PhysicalDomain=network_engine_domain  SubClassName=ps_output  LeftPortType=input  RightPortType=output  PseudoPeriodic=off  Frequencies=[]  VectorFormat=1-D array  Unit=N  AffineConversion=off
  PS-Simulink Converter2 : nesl_utility/PS-Simulink Converter  PhysicalDomain=network_engine_domain  SubClassName=ps_output  LeftPortType=input  RightPortType=output  PseudoPeriodic=off  Frequencies=[]  VectorFormat=1-D array  Unit=m/s  AffineConversion=off
  PS-Simulink Converter3 : nesl_utility/PS-Simulink Converter  PhysicalDomain=network_engine_domain  SubClassName=ps_output  LeftPortType=input  RightPortType=output  PseudoPeriodic=off  Frequencies=[]  VectorFormat=1-D array  Unit=m  AffineConversion=off
  Terminator : Terminator
  R : PMIOPort  Side=Left
  C : PMIOPort  Port=2  Side=Right
  Out Bus Element : Outport  VectorParamsAs1DForOutWhenUnconnected=off  PortName=meas  Element=FDamper
  Out Bus Element1 : Outport  VectorParamsAs1DForOutWhenUnconnected=off  PortName=meas  Element=FBumpstop
  Out Bus Element2 : Outport  VectorParamsAs1DForOutWhenUnconnected=off  PortName=meas  Element=xDamper
  Out Bus Element3 : Outport  VectorParamsAs1DForOutWhenUnconnected=off  PortName=meas  Element=vDamper
  wires:
  PS-Simulink Converter1/1 -> Out Bus Element1/1
  PS-Simulink Converter3/1 -> Out Bus Element2/1
  PS-Simulink Converter2/1 -> Out Bus Element3/1
  PS-Simulink Converter/1 -> Out Bus Element/1
  Ctrl/1 -> Terminator/1
  connections:
  R/RConn1 -- Motion Damper/LConn1 -- Bumpstop/LConn1 -- Damper/LConn1
  Force Damper/RConn1 -- Damper/RConn1
  Force Bumpstop/RConn1 -- Bumpstop/RConn1
  PS-Simulink Converter/LConn1 -- Force Damper/RConn2
  PS-Simulink Converter3/LConn1 -- Motion Damper/RConn3
  PS-Simulink Converter1/LConn1 -- Force Bumpstop/RConn2
  PS-Simulink Converter2/LConn1 -- Motion Damper/RConn2
  Force Damper/LConn1 -- C/RConn1 -- Force Bumpstop/LConn1 -- Motion Damper/RConn1

== system sm_car/Vehicle/Vehicle/Chassis/Damper/Decoupled/Damper A2 Heave/None ==
  note: Sensor inserted simply to ensure
      | all blocks are connected to a network
  Ctrl : Inport
  Constant{1..4} (4 alike) : Constant  Value=0
  Ideal Translational Motion Sensor : fl_lib/Mechanical/Mechanical Sensors/Ideal Translational Motion Sensor  reference=foundation.enum.MeasurementReference.difference  acceleration_port=false  velocity_port=true  position_port=true  offset=0 m
  PS-Simulink Converter2 : nesl_utility/PS-Simulink Converter  PhysicalDomain=network_engine_domain  SubClassName=ps_output  LeftPortType=input  RightPortType=output  PseudoPeriodic=off  Frequencies=[]  VectorFormat=1-D array  Unit=1  AffineConversion=off
  PS-Simulink Converter3 : nesl_utility/PS-Simulink Converter  PhysicalDomain=network_engine_domain  SubClassName=ps_output  LeftPortType=input  RightPortType=output  PseudoPeriodic=off  Frequencies=[]  VectorFormat=1-D array  Unit=1  AffineConversion=off
  Terminator : Terminator
  Terminator1 : Terminator
  Terminator2 : Terminator
  R : PMIOPort  Side=Left
  C : PMIOPort  Port=2  Side=Right
  Out Bus Element : Outport  VectorParamsAs1DForOutWhenUnconnected=off  PortName=meas  Element=FDamper
  Out Bus Element1 : Outport  VectorParamsAs1DForOutWhenUnconnected=off  PortName=meas  Element=FBumpstop
  Out Bus Element2 : Outport  VectorParamsAs1DForOutWhenUnconnected=off  PortName=meas  Element=xDamper
  Out Bus Element3 : Outport  VectorParamsAs1DForOutWhenUnconnected=off  PortName=meas  Element=vDamper
  wires:
  PS-Simulink Converter2/1 -> Terminator1/1
  PS-Simulink Converter3/1 -> Terminator2/1
  Constant2/1 -> Out Bus Element1/1
  Constant4/1 -> Out Bus Element2/1
  Constant3/1 -> Out Bus Element3/1
  Constant1/1 -> Out Bus Element/1
  Ctrl/1 -> Terminator/1
  connections:
  C/RConn1 -- Ideal Translational Motion Sensor/RConn1
  R/RConn1 -- Ideal Translational Motion Sensor/LConn1
  PS-Simulink Converter3/LConn1 -- Ideal Translational Motion Sensor/RConn3
  Ideal Translational Motion Sensor/RConn2 -- PS-Simulink Converter2/LConn1

== system sm_car/Vehicle/Vehicle/Chassis/Damper/Decoupled/Damper A2 Heave/Nonlinear ==
  note: Sensing
  Ctrl : Inport
  Bumpstop : fl_lib/Mechanical/Translational Elements/Translational Hard Stop  upper_bnd=bs_lim_upper m  lower_bnd=bs_lim_lower m  model=1  stiff_up=bs_k_upper N/m  stiff_low=bs_k_lower N/m  D_up=bs_b_upper N/(m/s)  D_low=bs_b_lower N/(m/s)  transition=bs_region m  coeff_rest=0.7  v_tol=0.001 m/s  f_tol=0.001 N  v_specify=off  v_priority=None  v=0 m/s  v_nominal_specify=off  v_nominal_value=1  v_nominal_unit=m/s  f_specify=off  f_priority=None  f=0 N  f_nominal_specify=off  f_nominal_value=1  f_nominal_unit=N  x_specify=off  x_priority=High  x=0 m  x_nominal_specify=off  x_nominal_value=1  x_nominal_unit=m  M_specify=off  M_priority=None  M=0
  Damper : sdl_lib/Couplings & Drives/Springs & Dampers/Nonlinear Translational Damper  parameterization=2  symmetry=1  coefficient_vector=[10, 0, 1, 0, .1] N/(m/s)  extension_coefficient_vector=[10, 0, 1, 0, .1] N/(m/s)  contraction_coefficient_vector=[100, -1, 10, 0, 0] N/(m/s)  velocity_vector=velocity_vector m/s  force_vector=force_vector N  interp_method=simscape.enum.interpolation.linear  extrap_method=simscape.enum.extrapolation.linear
      settings: InternalSimscapePortConfiguration="{\"Bottom\":[],\"Left\":[{\"id\":\"R\",\"label\":\"R\",\"type\":\"foundation.mechanical.translational.translational\"}],\"Right\":[{\"id\":\"C\",\"label\":\"C\",\"type\":\"foundation.mechanical.translational.translational\"}],\"Top\":[]}"
  Force Bumpstop : fl_lib/Mechanical/Mechanical Sensors/Ideal Force Sensor
  Force Damper : fl_lib/Mechanical/Mechanical Sensors/Ideal Force Sensor
  Motion Damper : fl_lib/Mechanical/Mechanical Sensors/Ideal Translational Motion Sensor  reference=foundation.enum.MeasurementReference.difference  acceleration_port=false  velocity_port=true  position_port=true  offset=dam_x0 m
  PS-Simulink Converter : nesl_utility/PS-Simulink Converter  PhysicalDomain=network_engine_domain  SubClassName=ps_output  LeftPortType=input  RightPortType=output  PseudoPeriodic=off  Frequencies=[]  VectorFormat=1-D array  Unit=N  AffineConversion=off
  PS-Simulink Converter1 : nesl_utility/PS-Simulink Converter  PhysicalDomain=network_engine_domain  SubClassName=ps_output  LeftPortType=input  RightPortType=output  PseudoPeriodic=off  Frequencies=[]  VectorFormat=1-D array  Unit=N  AffineConversion=off
  PS-Simulink Converter2 : nesl_utility/PS-Simulink Converter  PhysicalDomain=network_engine_domain  SubClassName=ps_output  LeftPortType=input  RightPortType=output  PseudoPeriodic=off  Frequencies=[]  VectorFormat=1-D array  Unit=m/s  AffineConversion=off
  PS-Simulink Converter3 : nesl_utility/PS-Simulink Converter  PhysicalDomain=network_engine_domain  SubClassName=ps_output  LeftPortType=input  RightPortType=output  PseudoPeriodic=off  Frequencies=[]  VectorFormat=1-D array  Unit=m  AffineConversion=off
  Terminator : Terminator
  R : PMIOPort  Side=Left
  C : PMIOPort  Port=2  Side=Right
  Out Bus Element : Outport  VectorParamsAs1DForOutWhenUnconnected=off  PortName=meas  Element=FDamper
  Out Bus Element1 : Outport  VectorParamsAs1DForOutWhenUnconnected=off  PortName=meas  Element=FBumpstop
  Out Bus Element2 : Outport  VectorParamsAs1DForOutWhenUnconnected=off  PortName=meas  Element=xDamper
  Out Bus Element3 : Outport  VectorParamsAs1DForOutWhenUnconnected=off  PortName=meas  Element=vDamper
  wires:
  Ctrl/1 -> Terminator/1
  PS-Simulink Converter/1 -> Out Bus Element/1
  PS-Simulink Converter2/1 -> Out Bus Element3/1
  PS-Simulink Converter3/1 -> Out Bus Element2/1
  PS-Simulink Converter1/1 -> Out Bus Element1/1
  connections:
  Motion Damper/RConn1 -- Force Bumpstop/LConn1 -- C/RConn1 -- Force Damper/LConn1
  PS-Simulink Converter2/LConn1 -- Motion Damper/RConn2
  PS-Simulink Converter1/LConn1 -- Force Bumpstop/RConn2
  PS-Simulink Converter3/LConn1 -- Motion Damper/RConn3
  PS-Simulink Converter/LConn1 -- Force Damper/RConn2
  Force Bumpstop/RConn1 -- Bumpstop/RConn1
  Damper/RConn1 -- Force Damper/RConn1
  Bumpstop/LConn1 -- Motion Damper/LConn1 -- R/RConn1 -- Damper/LConn1
